simulink model "cp5_ej2_simple"  (R2026a)
settings: Solver=VariableStepAuto  StopTime=60  MaxStep=0.01
libraries: slpidlib x1
settings Model: Creator=benja  LastModifiedBy=benja

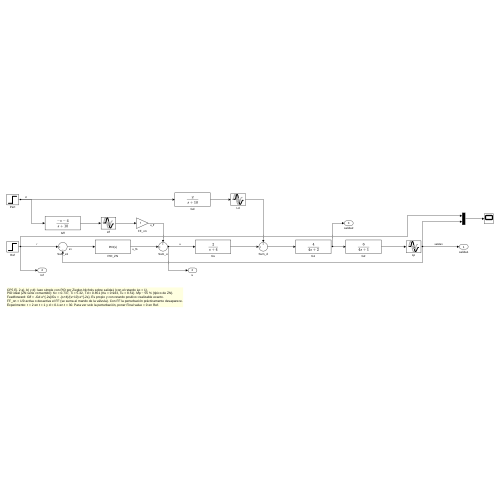
[thumbnail: Simulink's stored preview of the top-level diagram]
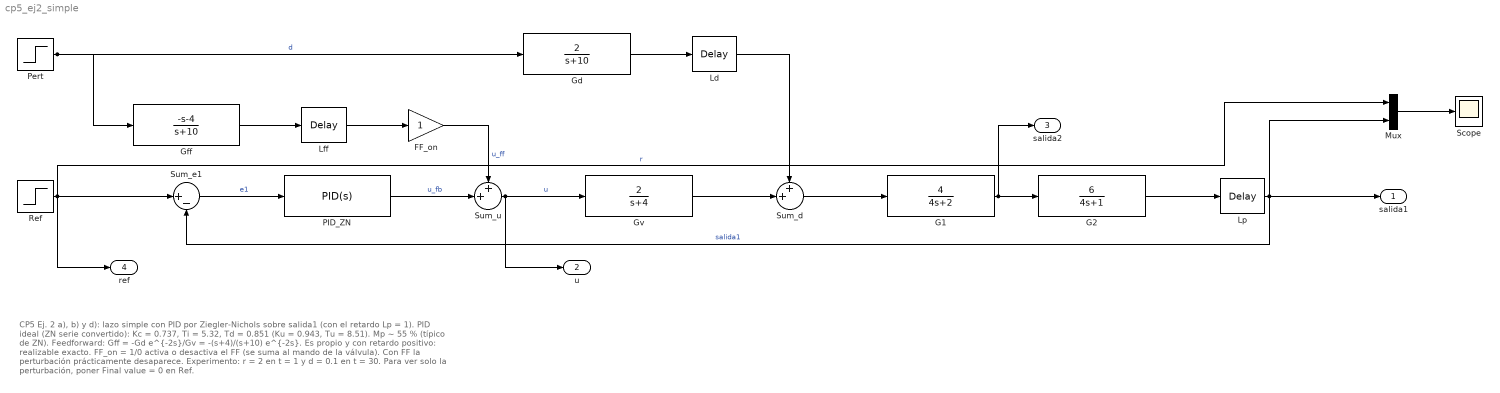
== system cp5_ej2_simple ==
  note: CP5 Ej. 2 a), b) y d): lazo simple con PID por Ziegler-Nichols sobre salida1 (con el retardo Lp = 1).
      | PID ideal (ZN serie convertido): Kc = 0.737, Ti = 5.32, Td = 0.851 (Ku = 0.943, Tu = 8.51). Mp ~ 55 % (típico de ZN).
      | Feedforward: Gff = -Gd e^{-2s}/Gv = -(s+4)/(s+10) e^{-2s}. Es propio y con retardo positivo: realizable exacto.
      | FF_on = 1/0 activa o desactiva el FF (se suma al mando de la válvula). Con FF la perturbación prácticamente desaparece.
      | Experimento: r = 2 en t = 1 y d = 0.1 en t = 30. Para ver solo la perturbación, poner Final value = 0 en Ref.
  FF_on : Gain
  G1 : TransferFcn  Numerator=4  Denominator=[4 2]
  G2 : TransferFcn  Numerator=6  Denominator=[4 1]
  Gd : TransferFcn  Numerator=2  Denominator=[1 10]
  Gff : TransferFcn  Numerator=[-1 -4]  Denominator=[1 10]
  Gv : TransferFcn  Numerator=2  Denominator=[1 4]
  Ld : TransportDelay  DelayTime=2
  Lff : TransportDelay  DelayTime=2
  Lp : TransportDelay
  Mux : Mux  Inputs=2
  PID_ZN : slpidlib/PID Controller  Controller=PID  Form=Ideal  TimeDomain=Continuous-time  UseExternalTs=off  SampleTime=-1  IntegratorMethod=Forward Euler  FilterMethod=Forward Euler  ControllerParametersSource=internal  P=0.7369  I=0.1881  UseKiTs=off  D=0.8506  UseExternalDerivativeSource=off  N=11.7571  UseFilter=on  TunerSelectOption=Transfer Function Based (PID Tuner App)  InitialConditionSource=internal  InitialConditionForIntegrator=0  InitialConditionForFilter=0  DifferentiatorICPrevScaledInput=0  ExternalReset=none  TrackingMode=off  Kt=1  LimitOutput=off  SatLimitsSource=internal  UpperSaturationLimit=inf  LowerSaturationLimit=-inf  LinearizeAsGain=on  AntiWindupMode=none  Kb=1  LimitIntegrator=off  UpperIntegratorSaturationLimit=inf  LowerIntegratorSaturationLimit=-inf  POutMin=[]  POutMax=[]  IOutMin=[]  IOutMax=[]  DOutMin=[]  DOutMax=[]  NOutMin=[]  NOutMax=[]  SumOutMin=[]  SumOutMax=[]  SaturationOutMin=[]  SaturationOutMax=[]  PParamMin=[]  PParamMax=[]  IParamMin=[]  IParamMax=[]  DParamMin=[]  DParamMax=[]  NParamMin=[]  NParamMax=[]  KbParamMin=[]  KbParamMax=[]  KtParamMin=[]  KtParamMax=[]  KbOutMin=[]  KbOutMax=[]  KtOutMin=[]  KtOutMax=[]  IntegratorOutMin=[]  IntegratorOutMax=[]  FilterOutMin=[]  FilterOutMax=[]  SumI1OutMin=[]  SumI1OutMax=[]  SumI2OutMin=[]  SumI2OutMax=[]  SumI3OutMin=[]  SumI3OutMax=[]  SumI4OutMin=[]  SumI4OutMax=[]  SumDOutMin=[]  SumDOutMax=[]  DifferentiatorOutMin=[]  DifferentiatorOutMax=[]  FilterDiffOutCoefMin=[]  FilterDiffOutCoefMax=[]  ReciprocalOutMin=[]  ReciprocalOutMax=[]  SumDenOutMin=[]  SumDenOutMax=[]  SumNumOutMin=[]  SumNumOutMax=[]  DivideOutMin=[]  DivideOutMax=[]  UdiffTsProdOutMin=[]  UdiffTsProdOutMax=[]  NTsProdOutMin=[]  NTsProdOutMax=[]  UintegralTsProdOutMin=[]  UintegralTsProdOutMax=[]  UngainTsProdOutMin=[]  UngainTsProdOutMax=[]  ClampingZeroOutDataTypeStr=Inherit: Inherit via back propagation  ClampingZeroOutMin=[]  ClampingZeroOutMax=[]  FilterDenConstantOutDataTypeStr=Inherit: Inherit via back propagation  FilterDenConstantOutMin=[]  FilterDenConstantOutMax=[]  PCopyOutDataTypeStr=Inherit: Inherit via back propagation  PCopyOutMin=[]  PCopyOutMax=[]  NCopyOutDataTypeStr=Inherit: Inherit via back propagation  NCopyOutMin=[]  NCopyOutMax=[]  IntegratorContinuousStateAttributes=''  IntegratorStateMustResolveToSignalObject=off  IntegratorRTWStateStorageClass=Auto  FilterContinuousStateAttributes=''  FilterStateMustResolveToSignalObject=off  FilterRTWStateStorageClass=Auto  ParallelPVariant=Passthrough  IdealPVariant=InternalParameters  IVariant=InternalParameters  DVariant=InternalParameters  IntegratorVariant=Continuous  SatVariant=Disabled  AWVariant=Passthrough  PCopyVariant=Disabled  TRVariant=Disabled  FdbkBlocksVariant=Forward  IdealPFdbkVariant=Disabled  SatFdbkVariant=Disabled  DerivativeFilterVariant=ContFilter  NVariant=InternalParameters  NCopyVariant=Disabled  FilterICVariant=InternalICsFilter  IntegratorICVariant=InternalICs  ExternalResetVariant=Disabled  TRSumVariant=Passthrough  SumFdbkVariant=Disabled  SumVariant=Sum_PID  TsampFilterVariant=InternalTs  TsampNgainVariant=Passthrough  TsampIntegralVariant=Disabled_SignalSpec  ExternalSaturationOutDataTypeStr=Inherit: Same as second input  DerivativeSourceVariant=ErrorSignal  PreIntVariant=InternalPreInt
  Pert : Step  Time=30  FinalValue=0.1  SampleTime=0
  Ref : Step  FinalValue=2  SampleTime=0
  Scope : Scope
  Sum_d : Sum  Inputs=++|
  Sum_e1 : Sum  Inputs=|+-
  Sum_u : Sum  Inputs=++|
  salida1 : Outport
  u : Outport  Port=2
  salida2 : Outport  Port=3
  ref : Outport  Port=4
  wires:
  Ref/1 -> Sum_e1/1, ref/1, Mux/1  "r"
  Sum_e1/1 -> PID_ZN/1  "e1"
  PID_ZN/1 -> Sum_u/2  "u_fb"
  Pert/1 -> Gff/1, Gd/1  "d"
  Gff/1 -> Lff/1
  Lff/1 -> FF_on/1
  FF_on/1 -> Sum_u/1  "u_ff"
  Sum_u/1 -> Gv/1, u/1  "u"
  Gv/1 -> Sum_d/2
  Gd/1 -> Ld/1
  Ld/1 -> Sum_d/1
  Sum_d/1 -> G1/1
  G1/1 -> G2/1, salida2/1
  G2/1 -> Lp/1
  Lp/1 -> salida1/1, Sum_e1/2, Mux/2  "salida1"
  Mux/1 -> Scope/1
